simulink model "HRES_ORC_PEM"  (R2025b)
settings: Solver=ode23t  StartTime=0.0  StopTime=35000  MaxStep=1728  RelTol=1e-3
model workspace (MAT data in the model file):
  CND_L = 10
  CND_T0 = 333.15
  CND_d = 0.012
  CND_n = 20
  CND_p0 = 150000
  GAS_Tmax = 430
  GAS_dT = 20
  GAS_kb = 0.04
  GAS_ki = 0.002
  GAS_kp = 0.05
  GAS_min = 0.02
  GAS_total = 5
  GAS_u0 = 0.05
  HRS_L = 10
  HRS_LG = 1
  HRS_d = 0.012
  HRS_n = 6
  HRS_nG = 25
  HRS_p0 = 0.3
  HRS_x0 = 0.2
  NOZ_kb = 0.025
  NOZ_ki = 0.0005
  NOZ_kp = 0.02
  NOZ_min = 0.01
  NOZ_u0 = 0.1
  ORC_T3set = 400
  ORC_Taux = -2
  ORC_Taux0 = 0
  ORC_kb = 0.4
  ORC_ki = 2e-07
  ORC_kp = 5e-07
  ORC_mdot0 = 0.2
  ORC_mmax = 1
  ORC_mmin = 0.01
  ORC_pset_MPa = 1
  RCV_V = 0.2
  RCV_frac0 = 0.5
  RCV_p0 = 0.15
  RCV_tau = 0.1
  TRB_Tref = 400
  TRB_mdot = 0.6
  TRB_pr = 6
values from neighbouring files (symbols this model uses):
  R_h2 = 4.12    [run_simulation.m]
libraries: fl_lib x62, nesl_utility x56, SimscapeFluids_lib x9, slpidlib x4, ee_lib x2
(part 1 of 5)
settings Model: Creator=moham  LastModifiedBy=moham
settings SolverCC: ZeroCrossAlgorithm=Adaptive
settings DebuggingCC: AlgebraicLoopMsg=none

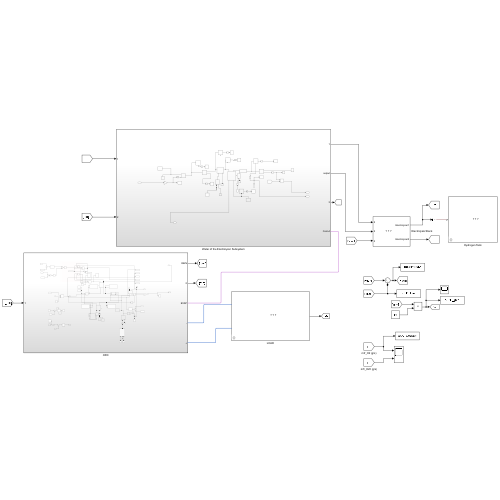
[thumbnail: Simulink's stored preview of the top-level diagram]
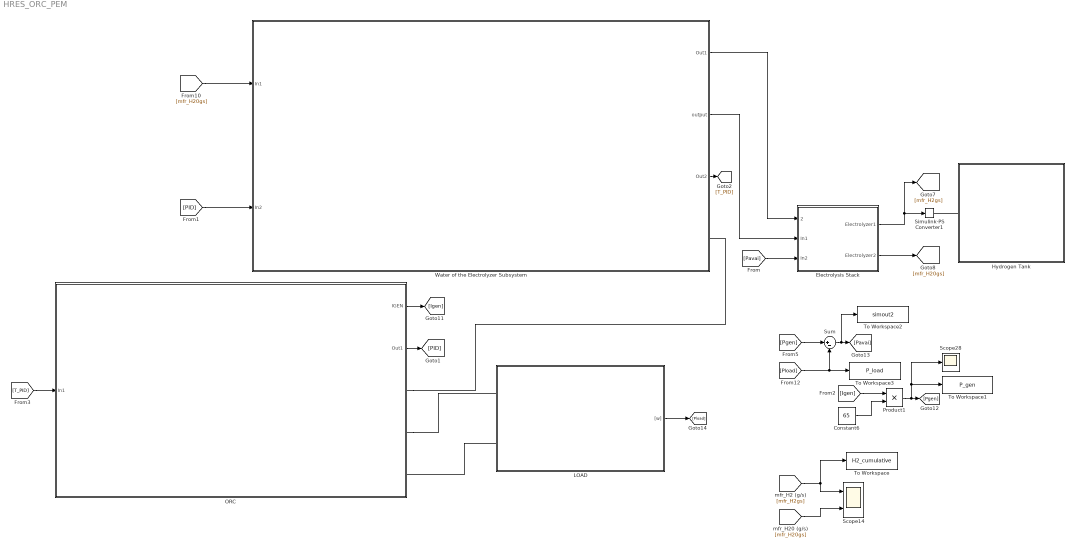
== system HRES_ORC_PEM ==
  Constant6 : Constant  Value=65
  "Electrolysis Stack " : Subsystem
      mask Display: image(imread("C:\Users\user\Desktop\workgrp2\1055082.png"));
  Hydrogen Tank : Subsystem
      mask Display: image(imread("C:\Users\user\Desktop\workgrp2\images.jpg"));
  LOAD : Subsystem
      mask Display: image(imread("C:\Users\user\Desktop\workgrp2\pngtree-factory-clipart-silhouette-png-image_2632918.jpg"));
  ORC : Subsystem
  Product1 : Product
  Scope14 : Scope  NumInputPorts=2
      settings: ActiveDisplayYMinimum=-0.021522256338686718  ActiveDisplayYMaximum=0.19369823375857767  DataLoggingVariableName=ScopeData14
  Scope28 : Scope
      settings: ActiveDisplayYMinimum=-3803.7118967481169  ActiveDisplayYMaximum=34231.003371105791  DataLoggingVariableName=ScopeData29
  Simulink-PS Converter1 : nesl_utility/Simulink-PS Converter  PhysicalDomain=network_engine_domain  SubClassName=ps_input  LeftPortType=input  RightPortType=output  PseudoPeriodic=off  Frequencies=[]  NoiseDistribution=none  NoiseParameters=[]  Unit=1  AffineConversion=off  FilteringAndDerivatives=provide  SimscapeFilterOrder=1  InputFilterTimeConstant=0.001  UdotUserProvided=0
  Sum : Sum  Inputs=|+-
  To Workspace : ToWorkspace  VariableName=H2_cumulative  SampleTime=-1
  To Workspace1 : ToWorkspace  VariableName=P_gen  SampleTime=-1
  To Workspace2 : ToWorkspace  VariableName=simout2  SampleTime=-1
  To Workspace3 : ToWorkspace  VariableName=P_load  SampleTime=-1
  Water of the Electrolyzer Subsystem : Subsystem
  wires:
  "Electrolysis Stack "/2(Electrolyzer2) -> [mfr_H20gs]
  [mfr_H20gs] -> Scope14/2
  [mfr_H2gs] -> Scope14/1, To Workspace/1
  "Electrolysis Stack "/1(Electrolyzer1) -> [mfr_H2gs], Simulink-PS Converter1/1
  [Igen] -> Product1/1
  Constant6/1 -> Product1/2
  Product1/1 -> To Workspace1/1, Scope28/1, [Pgen]
  [Pgen] -> Sum/1
  [Pload] -> Sum/2, To Workspace3/1
  Sum/1 -> To Workspace2/1, [Pavai]
  [Pavai] -> "Electrolysis Stack "/3(In2)
  LOAD/1("[w]") -> [Pload]
  [mfr_H20gs] -> Water of the Electrolyzer Subsystem/1(In1)
  Water of the Electrolyzer Subsystem/1(Out1) -> "Electrolysis Stack "/1(2)
  Water of the Electrolyzer Subsystem/2(output) -> "Electrolysis Stack "/2(In1)
  ORC/1(IGEN) -> [Igen]
  ORC/2(Out1) -> [PID]
  [PID] -> Water of the Electrolyzer Subsystem/2(In2)
  Water of the Electrolyzer Subsystem/3(Out2) -> [T_PID]
  [T_PID] -> ORC/1(In1)
  connections:
  Hydrogen Tank/LConn1 -- Simulink-PS Converter1/RConn1
  ORC/RConn1 -- Water of the Electrolyzer Subsystem/RConn1
  ORC/RConn2 -- LOAD/LConn1
  LOAD/LConn2 -- ORC/RConn3

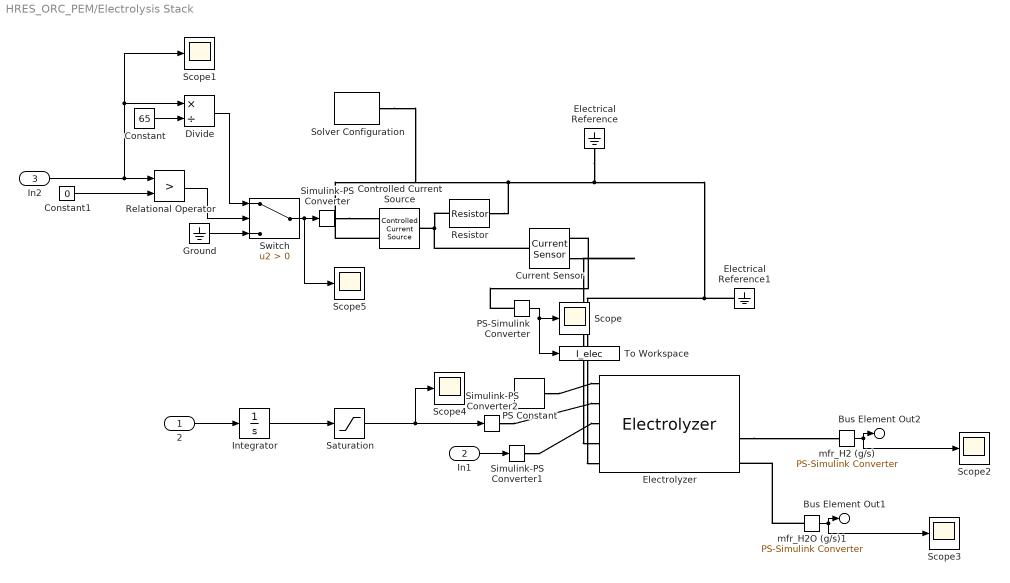
== system HRES_ORC_PEM/Electrolysis Stack  ==
  2 : Inport
  In1 : Inport  Port=2
  In2 : Inport  Port=3
  Constant : Constant  Value=65
  Constant1 : Constant  Value=0
  Controlled Current Source : fl_lib/Electrical/Electrical Sources/Controlled Current Source
  Current Sensor : fl_lib/Electrical/Electrical Sensors/Current Sensor
  Divide : Product  Inputs=*/
  Electrical Reference : fl_lib/Electrical/Electrical Elements/Electrical Reference
  Electrical Reference1 : fl_lib/Electrical/Electrical Elements/Electrical Reference
  Electrolyzer : ee_lib/Sources/Electrolyzer  pH_option=ee.enum.electrolyzer.pH.constant  R=0.1 Ohm  area=0.02 m^2  x=0.01 m  NCells=30  pH0=2.8  pHC=2.8  pH_vec=[5, 5.5, 6, 6.5, 7]  rho_vec=[.2, .75, 2.5, 8, 18.2] MOhm*cm  T_vec=[273, 298, 323, 348, 353.15] K  eff_vec=[0.75, 0.78, 0.80, 0.82, 0.85]  i_specify=off  i_priority=None  i=0 A  i_nominal_specify=off  i_nominal_value=1  i_nominal_unit=A  v_specify=off  v_priority=None  v=65 V  v_nominal_specify=off  v_nominal_value=1  v_nominal_unit=V  PE_specify=off  PE_priority=None  PE=100 J/s  PE_nominal_specify=off  PE_nominal_value=1  PE_nominal_unit=J/s  mol_e_specify=off  mol_e_priority=None  mol_e=1e3 mol/s  mol_e_nominal_specify=off  mol_e_nominal_value=1  mol_e_nominal_unit=mol/s  mol_h2_specify=off  mol_h2_priority=None  mol_h2=1e3 mol/s  mol_h2_nominal_specify=off  mol_h2_nominal_value=1  mol_h2_nominal_unit=mol/s  RT_specify=off  RT_priority=None  RT=1 Ohm  RT_nominal_specify=off  RT_nominal_value=1  RT_nominal_unit=Ohm  xhp_specify=off  xhp_priority=None  xhp=1 mol  xhp_nominal_specify=off  xhp_nominal_value=1  xhp_nominal_unit=mol
      settings: InternalSimscapePortConfiguration="{\"Bottom\":[],\"Left\":[{\"id\":\"purge\",\"label\":\"purge\",\"type\":\"input\"},{\"id\":\"vol\",\"label\":\"vol\",\"type\":\"input\"},{\"id\":\"T\",\"label\":\"T\",\"type\":\"input\"}],\"Right\":[{\"id\":\"volPurging\",\"label\":\"volPurging\",\"type\":\"output\"},{\"id\":\"pH\",\"label\":\"pH\",\"type\":\"output\"},{\"id\":\"mdotH2\",\"label\":\"mdotH2\",\"type\":\"output\"},{\"id\":\"mdotH2O\",\"label\":\"mdotH2O\",\"type\":\"output\"}],\"Top\":[{\"id\":\"p\",\"label\":\"+\",\"type\":\"foundation.electrical.electrical\"},{\"id\":\"n\",\"label\":\"-\",\"type\":\"foundation.electrical.electrical\"}]}"
  Ground : Ground
  Integrator : Integrator  InitialCondition=1e-3
  PS Constant : fl_lib/Physical Signals/Sources/PS Constant  constant=0
  PS-Simulink Converter : nesl_utility/PS-Simulink Converter  PhysicalDomain=network_engine_domain  SubClassName=ps_output  LeftPortType=input  RightPortType=output  PseudoPeriodic=off  Frequencies=[]  VectorFormat=inherit  Unit=inherit  AffineConversion=off
  Relational Operator : RelationalOperator  Operator=>  OutDataTypeStr=boolean  RndMeth=Simplest  InputSameDT=off
  Resistor : fl_lib/Electrical/Electrical Elements/Resistor  R=2000 Ohm  i_specify=off  i_priority=None  i=0 A  i_nominal_specify=off  i_nominal_value=1  i_nominal_unit=A  v_specify=off  v_priority=None  v=0 V  v_nominal_specify=off  v_nominal_value=1  v_nominal_unit=V
  Saturation : Saturate  UpperLimit=1.23  LowerLimit=0.1
  Scope{,1..5} (6 alike) : Scope
      Scope settings: ActiveDisplayYMinimum=-7.5063546369449288  ActiveDisplayYMaximum=67.5571917290874  DataLoggingVariableName=ScopeData5
      Scope1 settings: ActiveDisplayYMinimum=-640.94912444277657  ActiveDisplayYMaximum=4416.4653128627315  DataLoggingVariableName=ScopeData26
      Scope2 settings: ActiveDisplayYMinimum=-0.0023469124593997305  ActiveDisplayYMaximum=0.021122212133526698  DataLoggingVariableName=ScopeData7
      Scope3 settings: ActiveDisplayYMinimum=-0.020973427268130351  ActiveDisplayYMaximum=0.18876084540360316  DataLoggingVariableName=ScopeData3
      Scope4 settings: ActiveDisplayYMinimum=0.4  ActiveDisplayYMaximum=0.6  DataLoggingVariableName=ScopeData9
      Scope5 settings: DataLoggingVariableName=ScopeData31
  Simulink-PS Converter : nesl_utility/Simulink-PS Converter  PhysicalDomain=network_engine_domain  SubClassName=ps_input  LeftPortType=input  RightPortType=output  PseudoPeriodic=off  Frequencies=[]  NoiseDistribution=none  NoiseParameters=[]  Unit=1  AffineConversion=off  FilteringAndDerivatives=provide  SimscapeFilterOrder=1  InputFilterTimeConstant=0.001  UdotUserProvided=0
  Simulink-PS Converter1 : nesl_utility/Simulink-PS Converter  PhysicalDomain=network_engine_domain  SubClassName=ps_input  LeftPortType=input  RightPortType=output  PseudoPeriodic=off  Frequencies=[]  NoiseDistribution=none  NoiseParameters=[]  Unit=K  AffineConversion=off  FilteringAndDerivatives=provide  SimscapeFilterOrder=1  InputFilterTimeConstant=0.001  UdotUserProvided=0
  Simulink-PS Converter2 : nesl_utility/Simulink-PS Converter  PhysicalDomain=network_engine_domain  SubClassName=ps_input  LeftPortType=input  RightPortType=output  PseudoPeriodic=off  Frequencies=[]  NoiseDistribution=none  NoiseParameters=[]  Unit=1  AffineConversion=off  FilteringAndDerivatives=provide  SimscapeFilterOrder=1  InputFilterTimeConstant=0.001  UdotUserProvided=0
  Solver Configuration : nesl_utility/Solver Configuration  PhysicalDomain=network_engine_domain  SubClassName=solver  LeftPortType=input  RightPortType=generic  Tones=[]  Harmonics=[]  SimulateNoise=off  Profile=off  UseLocalSampling=off  EnableSwitchedLinearOptims=on  FrequencyDomain=off  UseCCode=off  RelTol=0.001  AbsTol=0.001  MinStep=1e-09  ToWorkspace=off  RevertToSquareIcSolve=off  NumHomotopyIterations=100  PhasorMode=off  PhasorModeNumHarmonics=1  ConsistencySolver=NEWTON_XTOL_AFTER_FTOL  IndexReductionMethod=DerivativeReplacement  DoDC=off  ResidualTolerance=1e-09  ConsistencyTolSource=GLOBAL  ConsistencyAbsTol=0.001  ConsistencyRelTol=0.001  ConsistencyTolFactor=0.001  UseLocalSolver=off  LocalSolverChoice=NE_BACKWARD_EULER_ADVANCER  ResolveIndetEquations=on  FunctionEvalNumThread=1  LocalSolverSampleTime=0.001  DoFixedCost=off  MaxNonlinIter=3  MaxModeIter=2  ComputeImpulses=off  ImpulseIterations=2  LinearAlgebra=auto  LinearAlgebraNumThread=0  EquationFormulation=NE_TIME_EF  DelaysMemoryBudget=1024  AutomaticFiltering=on  FilteringTimeConstant=0.001  PartitionStorageMethod=AS_NEEDED  PartitionMemoryBudget=1024  PartitionMethod=ROBUST  MultibodyUseLocalSolver=off  MultibodyLocalSolverChoice=ODE1  MultibodyLocalSolverSampleTime=0.001
  Switch : Switch  Criteria=u2 > Threshold  SaturateOnIntegerOverflow=off  InputSameDT=off
  To Workspace : ToWorkspace  VariableName=I_elec  SampleTime=-1
  mfr_H2 (g/s) : nesl_utility/PS-Simulink Converter  PhysicalDomain=network_engine_domain  SubClassName=ps_output  LeftPortType=input  RightPortType=output  PseudoPeriodic=off  Frequencies=[]  VectorFormat=inherit  Unit=g/s  AffineConversion=off
  mfr_H2O (g/s)1 : nesl_utility/PS-Simulink Converter  PhysicalDomain=network_engine_domain  SubClassName=ps_output  LeftPortType=input  RightPortType=output  PseudoPeriodic=off  Frequencies=[]  VectorFormat=inherit  Unit=g/s  AffineConversion=off
  Bus Element Out2 : Outport  PortName=Electrolyzer1  Element=H2_mfr(g/s)
  Bus Element Out1 : Outport  Port=2  PortName=Electrolyzer2  Element=H2O_mfr(g/s)
  wires:
  PS-Simulink Converter/1 -> Scope/1, To Workspace/1
  mfr_H2 (g/s)/1 -> Scope2/1, Bus Element Out2/1
  mfr_H2O (g/s)1/1 -> Scope3/1, Bus Element Out1/1
  In1/1 -> Simulink-PS Converter1/1
  Saturation/1 -> Scope4/1, Simulink-PS Converter2/1
  Ground/1 -> Switch/3
  Relational Operator/1 -> Switch/2
  Constant/1 -> Divide/2
  Constant1/1 -> Relational Operator/2
  Divide/1 -> Switch/1
  In2/1 -> Scope1/1, Divide/1, Relational Operator/1
  Switch/1 -> Scope5/1, Simulink-PS Converter/1
  2/1 -> Integrator/1
  Integrator/1 -> Saturation/1
  connections:
  Electrical Reference/LConn1 -- Resistor/RConn1 -- Controlled Current Source/RConn2 -- Solver Configuration/RConn1 -- Electrolyzer/LConn5 -- Electrical Reference1/LConn1
  PS-Simulink Converter/LConn1 -- Current Sensor/RConn1
  PS Constant/RConn1 -- Electrolyzer/LConn1
  Resistor/LConn1 -- Current Sensor/LConn1 -- Controlled Current Source/LConn1
  Electrolyzer/RConn3 -- mfr_H2 (g/s)/LConn1
  mfr_H2O (g/s)1/LConn1 -- Electrolyzer/RConn4
  Simulink-PS Converter1/RConn1 -- Electrolyzer/LConn3
  Simulink-PS Converter2/RConn1 -- Electrolyzer/LConn2
  Current Sensor/RConn2 -- Electrolyzer/LConn4
  Simulink-PS Converter/RConn1 -- Controlled Current Source/RConn1
